simulink subsystem "SunDirection"  (R2024b)
settings: Solver=VariableStepAuto  StartTime=0.0  StopTime=10.0  RelTol=1e-3
settings Model: Creator=marco  LastModifiedBy=marco

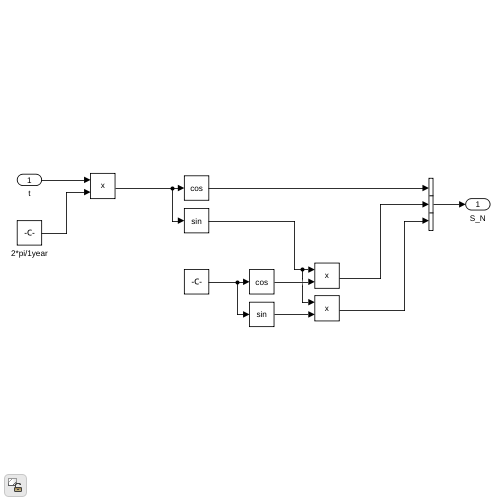
[thumbnail: Simulink's stored preview of the top-level diagram]
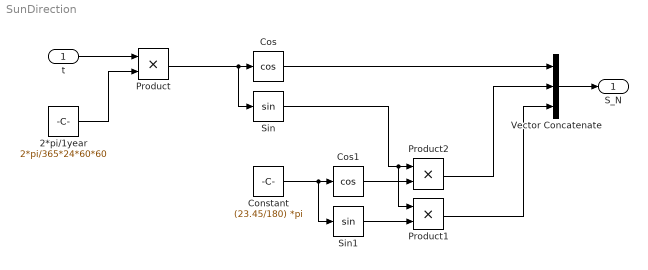
== system SunDirection ==
  t : Inport
  2*pi/1year : Constant  Value=2*pi/365*24*60*60
  Constant : Constant  Value=(23.45/180) *pi
  Cos : Trigonometry  Operator=cos
  Cos1 : Trigonometry  Operator=cos
  Product : Product
  Product1 : Product
  Product2 : Product
  Sin : Trigonometry
  Sin1 : Trigonometry
  Vector Concatenate : Concatenate  NumInputs=3
  S_N : Outport
  wires:
  2*pi/1year/1 -> Product/2
  Vector Concatenate/1 -> S_N/1
  Product1/1 -> Vector Concatenate/3
  Product2/1 -> Vector Concatenate/2
  Cos/1 -> Vector Concatenate/1
  Sin/1 -> Product1/1, Product2/1
  Sin1/1 -> Product1/2
  Cos1/1 -> Product2/2
  Constant/1 -> Sin1/1, Cos1/1
  Product/1 -> Sin/1, Cos/1
  t/1 -> Product/1
